simulink model "HorizontalClosedLoop"  (R2026b)
settings: Solver=FixedStepDiscrete  StopTime=25  FixedStep=.0025
undefined symbols (not defined in the file): Official
libraries: slpidlib x7
(part 1 of 3)
settings Model: Creator=tyasukaw  LastModifiedBy=tyasukaw

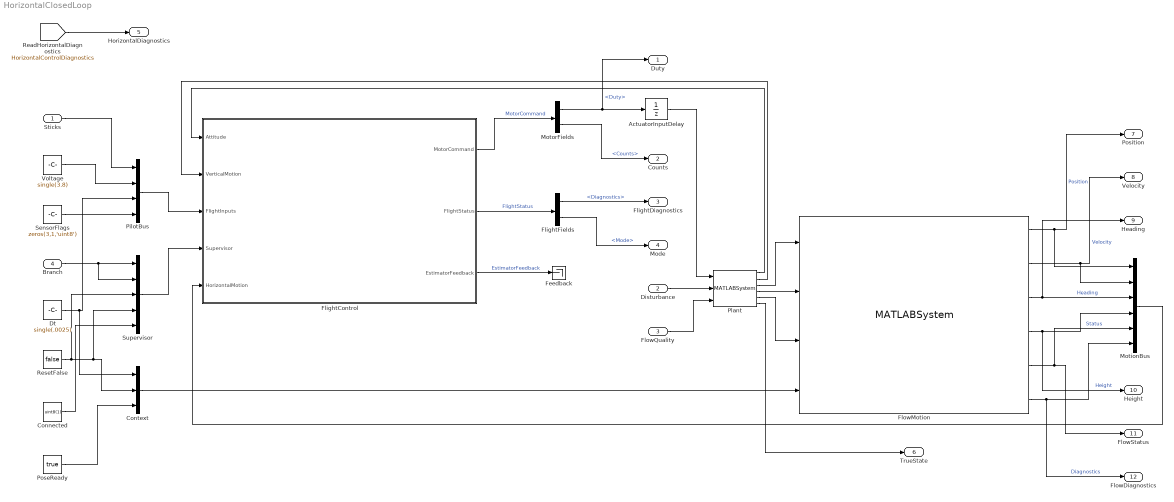
== system HorizontalClosedLoop ==
  Sticks : Inport  OutDataTypeStr=single  PortDimensions=6  SampleTime=.0025
  Disturbance : Inport  Port=2  OutDataTypeStr=single  PortDimensions=2  SampleTime=.0025
  FlowQuality : Inport  Port=3  OutDataTypeStr=uint16  SampleTime=.0025
  Branch : Inport  Port=4  OutDataTypeStr=uint8  SampleTime=.0025
  ActuatorInputDelay : UnitDelay  InitialCondition=zeros(4,1,'single')  SampleTime=.0025
  Connected : Constant  Value=uint8(1)
  Context : BusCreator  Inputs=3  OutDataTypeStr=Bus: HorizontalContextBus  NonVirtualBus=on
      settings: InheritFromInputs=off
  Dt : Constant  Value=single(.0025)
  Feedback : Terminator
  FlightControl : Subsystem  Description=最上位 Stateflow の指令と姿勢・高度を受け、離着陸、7 個の PID、モーター配分を計算します。出力は Duty・PWM Counts、飛行状態、次周期の推定器コンテキストです。状態ログもこの階層に含みます。
      mask help: 最上位 Stateflow の指令と姿勢・高度を受け、離着陸、7 個の PID、モーター配分を計算します。出力は Duty・PWM Counts、飛行状態、次周期の推定器コンテキストです。状態ログもこの階層に含みます。
      mask Display: disp('FlightControl');port_label('input',1,'Attitude');port_label('input',2,'VerticalMotion');port_label('input',3,'FlightInputs');port_label('input',4,'Supervisor');port_label('input',5,'HorizontalMotion');port_label('output',1,'MotorCommand');port_label('output',2,'FlightStatus');port_label('output',3,'EstimatorFeedback');
  FlightFields : BusSelector  OutputSignals=Diagnostics,Mode
  FlowMotion : MATLABSystem  Description=|  System=horizontal.FlowMotion  SampleTime=.0025  WindowSamples=8  XCountsPerRad=385  YCountsPerRad=385  MinQuality=25  MinHeightM=.12  MaxHeightM=1.0  MaxRangeAgeS=.15  MaxFlowAgeS=.025  MaxSampleGapS=.01  MaxGyroAgeS=.0075  MaxSpeedMps=1.5  MaxVerticalSpeedMps=2.0  MaxTiltDeg=25  VelocityTimeConstantS=.05  SimulateUsing=Code generation
      | %FLOWMOTION 概要：400 Hzの光学フロー・角速度を同一区間で集計し、
      |     % 50 Hzで水平速度と相対位置を推定します。局所Xは基準機首、Yは右。
      |     % 不良区間を速度ゼロに置き換えず、Statusで使用可否を公開します。
      mask Type: horizontal.FlowMotion
  MotionBus : BusCreator  Inputs=6  OutDataTypeStr=Bus: HorizontalMotionBus  NonVirtualBus=on
      settings: InheritFromInputs=off
  MotorFields : BusSelector  OutputSignals=Duty,Counts
  PilotBus : BusCreator  Inputs=4  OutDataTypeStr=Bus: HorizontalTestPilotBus  NonVirtualBus=on
      settings: InheritFromInputs=off
  Plant : MATLABSystem  System=horizontaltest.Plant  SampleTime=.0025  HoverDuty=.659  MotorLagS=.04  LinearDampingPerS=.5  TorqueAccelPerCount=.15  AngularDampingPerS=4  RangeDelayS=.035  FlowScale=1  GyroDelayS=0  HeadingDriftDegps=0  SimulateUsing=Code generation
      mask Type: horizontaltest.Plant
  PoseReady : Constant  Value=true
  ResetFalse : Constant  Value=false
  SensorFlags : Constant  Value=zeros(3,1,'uint8')
  Supervisor : BusCreator  Inputs=5  OutDataTypeStr=Bus: HorizontalTestSupervisorBus  NonVirtualBus=on
      settings: InheritFromInputs=off
  Voltage : Constant  Value=single(3.8)
  Duty : Outport
  Counts : Outport  Port=2
  FlightDiagnostics : Outport  Port=3
  Mode : Outport  Port=4
  HorizontalDiagnostics : Outport  Port=5
  TrueState : Outport  Port=6
  Position : Outport  Port=7
  Velocity : Outport  Port=8
  Heading : Outport  Port=9
  Height : Outport  Port=10
  FlowStatus : Outport  Port=11
  FlowDiagnostics : Outport  Port=12
  wires:
  Plant/6 -> TrueState/1
  [HorizontalControlDiagnostics] -> HorizontalDiagnostics/1
  FlightFields/2 -> Mode/1  "<Mode>"
  FlightFields/1 -> FlightDiagnostics/1  "<Diagnostics>"
  MotorFields/2 -> Counts/1  "<Counts>"
  FlowMotion/6 -> MotionBus/6, FlowDiagnostics/1  "Diagnostics"
  FlowMotion/5 -> MotionBus/5, FlowStatus/1  "Status"
  FlowMotion/4 -> MotionBus/4, Height/1  "Height"
  FlowMotion/3 -> MotionBus/3, Heading/1  "Heading"
  FlowMotion/2 -> MotionBus/2, Velocity/1  "Velocity"
  FlowMotion/1 -> MotionBus/1, Position/1  "Position"
  FlightControl/3(EstimatorFeedback) -> Feedback/1  "EstimatorFeedback"
  FlightControl/2(FlightStatus) -> FlightFields/1  "FlightStatus"
  PoseReady/1 -> Context/3
  Connected/1 -> Supervisor/5
  ResetFalse/1 -> Supervisor/4, Context/2, Supervisor/3
  Branch/1 -> Supervisor/1, Supervisor/2
  SensorFlags/1 -> PilotBus/4
  Dt/1 -> PilotBus/3, Context/1
  Voltage/1 -> PilotBus/2
  Sticks/1 -> PilotBus/1
  Context/1 -> FlowMotion/4
  Plant/5 -> FlowMotion/3
  Plant/4 -> FlowMotion/2
  Plant/3 -> FlowMotion/1
  FlowQuality/1 -> Plant/3
  Disturbance/1 -> Plant/2
  ActuatorInputDelay/1 -> Plant/1
  MotorFields/1 -> ActuatorInputDelay/1, Duty/1  "<Duty>"
  FlightControl/1(MotorCommand) -> MotorFields/1  "MotorCommand"
  MotionBus/1 -> FlightControl/5(HorizontalMotion)
  Supervisor/1 -> FlightControl/4(Supervisor)
  PilotBus/1 -> FlightControl/3(FlightInputs)
  Plant/2 -> FlightControl/2(VerticalMotion)
  Plant/1 -> FlightControl/1(Attitude)

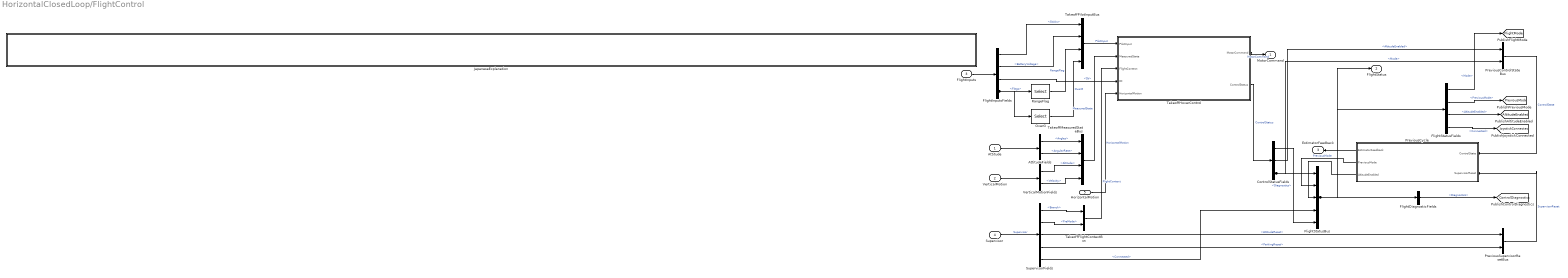
== system HorizontalClosedLoop/FlightControl ==
  Attitude : Inport
  VerticalMotion : Inport  Port=2
  FlightInputs : Inport  Port=3
  Supervisor : Inport  Port=4
  HorizontalMotion : Inport  Description=HorizontalMotion：水平推定・制御のデータと実行条件を選択・結合します。2軸の順序は局所X（基準機首）、Y（右）です。  Port=5  OutDataTypeStr=Bus: HorizontalMotionBus
  AttitudeFields : BusSelector  Description=AttitudeFields：バスから Angles,AngularRate を選びます。元のベクトルの成分順序は変更しません。  OutputSignals=Angles,AngularRate
  ControlStatusFields : BusSelector  Description=ControlStatusFields：バスから Diagnostics,AltitudeEnabled,Mode を選びます。元のベクトルの成分順序は変更しません。  OutputSignals=Diagnostics,AltitudeEnabled,Mode
  FlightDiagnosticFields : BusSelector  Description=FlightDiagnosticFields：バスから Diagnostics を選びます。元のベクトルの成分順序は変更しません。  OutputSignals=Diagnostics
  FlightInputsFields : BusSelector  Description=FlightInputsFields：バスから Sticks,BatteryVoltage,Dt,Flags を選びます。元のベクトルの成分順序は変更しません。  OutputSignals=Sticks,BatteryVoltage,Dt,Flags
  FlightStatusBus : BusCreator  Description=FlightStatusBus：異なる単位・型を持つ関連信号を名前付きバスにまとめます。入力線の信号名が項目名です。  Inputs=5
  FlightStatusFields : BusSelector  Description=FlightStatusFields：バスから Mode,PreviousMode,AltitudeEnabled,Connected を選びます。元のベクトルの成分順序は変更しません。  OutputSignals=Mode,PreviousMode,AltitudeEnabled,Connected
  JapaneseExplanation : Subsystem  Description=最上位 Stateflow の指令と姿勢・高度を受け、離着陸、7 個の PID、モーター配分を計算します。出力は Duty・PWM Counts、飛行状態、次周期の推定器コンテキストです。状態ログもこの階層に含みます。
      mask help: 最上位 Stateflow の指令と姿勢・高度を受け、離着陸、7 個の PID、モーター配分を計算します。出力は Duty・PWM Counts、飛行状態、次周期の推定器コンテキストです。状態ログもこの階層に含みます。
      mask Display: disp(sprintf('最上位 Stateflow の指令と姿勢・高度を受け、離着陸、7 個の PID、モーター配分を計算します。\n出力は Duty・PWM Counts、飛行状態、次周期の推定器コンテキストです。\n状態ログもこの階層に含みます。'));
  OverG : Selector  Description=OverG：必要なベクトル成分を選びます。選択位置は設定画面の Indices で確認します。  InputPortWidth=3  IndexOptions=Index vector (dialog)  Indices=1  OutputSizes=1
  PreviousControlStateBus : BusCreator  Description=PreviousControlStateBus：異なる単位・型を持つ関連信号を名前付きバスにまとめます。入力線の信号名が項目名です。  Inputs=2
  PreviousCycle : Subsystem  Description=前周期の推力・指令・モードなどを保持し、制御と次周期フィードバックへ渡します。Unit Delay は既存の更新順序を保つために必要です。
      mask help: 前周期の推力・指令・モードなどを保持し、制御と次周期フィードバックへ渡します。Unit Delay は既存の更新順序を保つために必要です。
      mask Display: disp('PreviousCycle');port_label('input',1,'ControlState');port_label('input',2,'SupervisorReset');port_label('output',1,'EstimatorFeedback');port_label('output',2,'PreviousMode');port_label('output',3,'AltitudeEnabled');
  PreviousSupervisorResetBus : BusCreator  Description=PreviousSupervisorResetBus：異なる単位・型を持つ関連信号を名前付きバスにまとめます。入力線の信号名が項目名です。  Inputs=2
  RangeFlag : Selector  Description=RangeFlag：必要なベクトル成分を選びます。選択位置は設定画面の Indices で確認します。  InputPortWidth=3  IndexOptions=Index vector (dialog)  Indices=2  OutputSizes=1
  SupervisorFields : BusSelector  Description=SupervisorFields：バスから Branch,PreMode,AttitudeReset,ParkingReset,Connected を選びます。元のベクトルの成分順序は変更しません。  OutputSignals=Branch,PreMode,AttitudeReset,ParkingReset,Connected
  TakeoffFlightContextBus : BusCreator  Description=TakeoffFlightContextBus：異なる単位・型を持つ関連信号を名前付きバスにまとめます。入力線の信号名が項目名です。  Inputs=2
  TakeoffHoverControl : Subsystem  Description=離着陸・高度制御・姿勢制御・角速度制御・モーター配分を機能別にまとめます。高度→速度、角度→角速度の二重ループを読みます。
      mask help: 離着陸・高度制御・姿勢制御・角速度制御・モーター配分を機能別にまとめます。高度→速度、角度→角速度の二重ループを読みます。
      mask Display: disp('TakeoffHoverControl');port_label('input',1,'PilotInput');port_label('input',2,'MeasuredState');port_label('input',3,'FlightContext');port_label('input',4,'Dt');port_label('input',5,'HorizontalMotion');port_label('output',1,'MotorCommand');port_label('output',2,'ControlStatus');
  TakeoffMeasuredStateBus : BusCreator  Description=TakeoffMeasuredStateBus：異なる単位・型を持つ関連信号を名前付きバスにまとめます。入力線の信号名が項目名です。  Inputs=4
  TakeoffPilotInputBus : BusCreator  Description=TakeoffPilotInputBus：異なる単位・型を持つ関連信号を名前付きバスにまとめます。入力線の信号名が項目名です。  Inputs=4
  VerticalMotionFields : BusSelector  Description=VerticalMotionFields：バスから Altitude,Velocity を選びます。元のベクトルの成分順序は変更しません。  OutputSignals=Altitude,Velocity
  MotorCommand : Outport
  FlightStatus : Outport  Port=2
  EstimatorFeedback : Outport  Port=3
  tag scope: AltitudeEnabled=global, ControlDiagnostics=global, FlightMode=global, JoystickConnected=global, PreviousMode=global
  wires:
  PreviousControlStateBus/1 -> PreviousCycle/1(ControlState)  "ControlState"
  FlightStatusFields/3 -> [AltitudeEnabled]  "<AltitudeEnabled>"
  PreviousCycle/1(EstimatorFeedback) -> EstimatorFeedback/1
  PreviousCycle/2(PreviousMode) -> FlightStatusBus/2  "PreviousMode"
  FlightStatusFields/1 -> [FlightMode]  "<Mode>"
  PreviousCycle/3(AltitudeEnabled) -> FlightStatusBus/3
  FlightStatusFields/2 -> [PreviousMode]  "<PreviousMode>"
  FlightStatusBus/1 -> FlightStatusFields/1, FlightDiagnosticFields/1, FlightStatus/1
  ControlStatusFields/3 -> FlightStatusBus/1, PreviousControlStateBus/2  "<Mode>"
  ControlStatusFields/1 -> FlightStatusBus/5  "<Diagnostics>"
  TakeoffHoverControl/1(MotorCommand) -> MotorCommand/1  "MotorCommand"
  HorizontalMotion/1 -> TakeoffHoverControl/5(HorizontalMotion)  "HorizontalMotion"
  TakeoffMeasuredStateBus/1 -> TakeoffHoverControl/2(MeasuredState)  "MeasuredState"
  TakeoffFlightContextBus/1 -> TakeoffHoverControl/3(FlightContext)  "FlightContext"
  TakeoffPilotInputBus/1 -> TakeoffHoverControl/1(PilotInput)  "PilotInput"
  SupervisorFields/5 -> FlightStatusBus/4  "<Connected>"
  SupervisorFields/4 -> PreviousSupervisorResetBus/2  "<ParkingReset>"
  SupervisorFields/3 -> PreviousSupervisorResetBus/1  "<AttitudeReset>"
  PreviousSupervisorResetBus/1 -> PreviousCycle/2(SupervisorReset)  "SupervisorReset"
  SupervisorFields/2 -> TakeoffFlightContextBus/2  "<PreMode>"
  SupervisorFields/1 -> TakeoffFlightContextBus/1  "<Branch>"
  TakeoffHoverControl/2(ControlStatus) -> ControlStatusFields/1  "ControlStatus"
  AttitudeFields/2 -> TakeoffMeasuredStateBus/2  "<AngularRate>"
  AttitudeFields/1 -> TakeoffMeasuredStateBus/1  "<Angles>"
  VerticalMotionFields/1 -> TakeoffMeasuredStateBus/3  "<Altitude>"
  OverG/1 -> TakeoffPilotInputBus/4  "OverG"
  RangeFlag/1 -> TakeoffPilotInputBus/3  "RangeFlag"
  VerticalMotionFields/2 -> TakeoffMeasuredStateBus/4  "<Velocity>"
  FlightInputsFields/2 -> TakeoffPilotInputBus/2  "<BatteryVoltage>"
  FlightInputsFields/4 -> OverG/1, RangeFlag/1  "<Flags>"
  FlightInputsFields/1 -> TakeoffPilotInputBus/1  "<Sticks>"
  FlightStatusFields/4 -> [JoystickConnected]  "<Connected>"
  FlightInputsFields/3 -> TakeoffHoverControl/4(Dt)  "<Dt>"
  FlightInputs/1 -> FlightInputsFields/1
  FlightDiagnosticFields/1 -> [ControlDiagnostics]  "<Diagnostics>"
  Attitude/1 -> AttitudeFields/1
  ControlStatusFields/2 -> PreviousControlStateBus/1  "<AltitudeEnabled>"
  VerticalMotion/1 -> VerticalMotionFields/1
  Supervisor/1 -> SupervisorFields/1  "Supervisor"

== system HorizontalClosedLoop/FlightControl/JapaneseExplanation ==

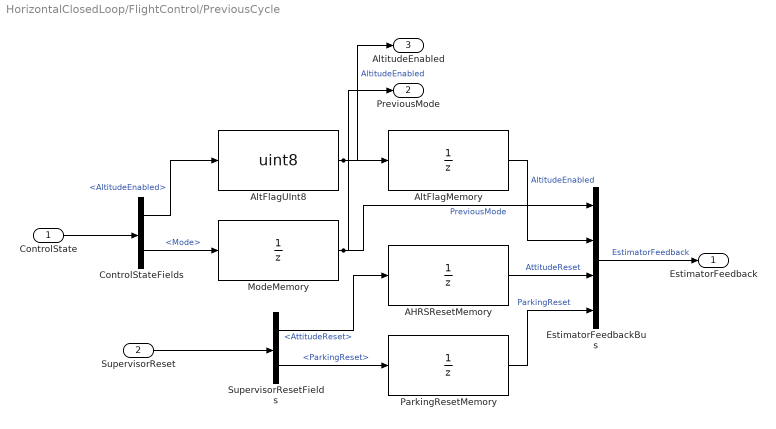
== system HorizontalClosedLoop/FlightControl/PreviousCycle ==
  ControlState : Inport
  SupervisorReset : Inport  Port=2
  AHRSResetMemory : UnitDelay  Description=AHRSResetMemory：前周期の値を保持して出力します。更新順序と状態保持に必要な 1 周期遅延です。初期値 false、周期 Official.Step 秒。  InitialCondition=false  SampleTime=Official.Step
  AltFlagMemory : UnitDelay  Description=AltFlagMemory：前周期の値を保持して出力します。更新順序と状態保持に必要な 1 周期遅延です。初期値 uint8(0)、周期 Official.Step 秒。  InitialCondition=uint8(0)  SampleTime=Official.Step
  AltFlagUInt8 : DataTypeConversion  Description=AltFlagUInt8：後段のバス・演算に合わせて uint8 型へ変換します。  OutDataTypeStr=uint8  SaturateOnIntegerOverflow=off  RndMeth=Floor
  ControlStateFields : BusSelector  Description=ControlStateFields：バスから AltitudeEnabled,Mode を選びます。元のベクトルの成分順序は変更しません。  OutputSignals=AltitudeEnabled,Mode
  EstimatorFeedbackBus : BusCreator  Description=EstimatorFeedbackBus：異なる単位・型を持つ関連信号を名前付きバスにまとめます。入力線の信号名が項目名です。  Inputs=4
  ModeMemory : UnitDelay  Description=ModeMemory：前周期の値を保持して出力します。更新順序と状態保持に必要な 1 周期遅延です。初期値 uint8(0)、周期 Official.Step 秒。  InitialCondition=uint8(0)  SampleTime=Official.Step
  ParkingResetMemory : UnitDelay  Description=ParkingResetMemory：前周期の値を保持して出力します。更新順序と状態保持に必要な 1 周期遅延です。初期値 false、周期 Official.Step 秒。  InitialCondition=false  SampleTime=Official.Step
  SupervisorResetFields : BusSelector  Description=SupervisorResetFields：バスから AttitudeReset,ParkingReset を選びます。元のベクトルの成分順序は変更しません。  OutputSignals=AttitudeReset,ParkingReset
  EstimatorFeedback : Outport
  PreviousMode : Outport  Port=2
  AltitudeEnabled : Outport  Port=3
  wires:
  AHRSResetMemory/1 -> EstimatorFeedbackBus/3  "AttitudeReset"
  EstimatorFeedbackBus/1 -> EstimatorFeedback/1  "EstimatorFeedback"
  AltFlagUInt8/1 -> AltitudeEnabled/1, AltFlagMemory/1  "AltitudeEnabled"
  ParkingResetMemory/1 -> EstimatorFeedbackBus/4  "ParkingReset"
  SupervisorResetFields/2 -> ParkingResetMemory/1  "<ParkingReset>"
  ControlStateFields/2 -> ModeMemory/1  "<Mode>"
  ControlState/1 -> ControlStateFields/1
  SupervisorReset/1 -> SupervisorResetFields/1
  ModeMemory/1 -> PreviousMode/1, EstimatorFeedbackBus/1  "PreviousMode"
  AltFlagMemory/1 -> EstimatorFeedbackBus/2  "AltitudeEnabled"
  SupervisorResetFields/1 -> AHRSResetMemory/1  "<AttitudeReset>"
  ControlStateFields/1 -> AltFlagUInt8/1  "<AltitudeEnabled>"

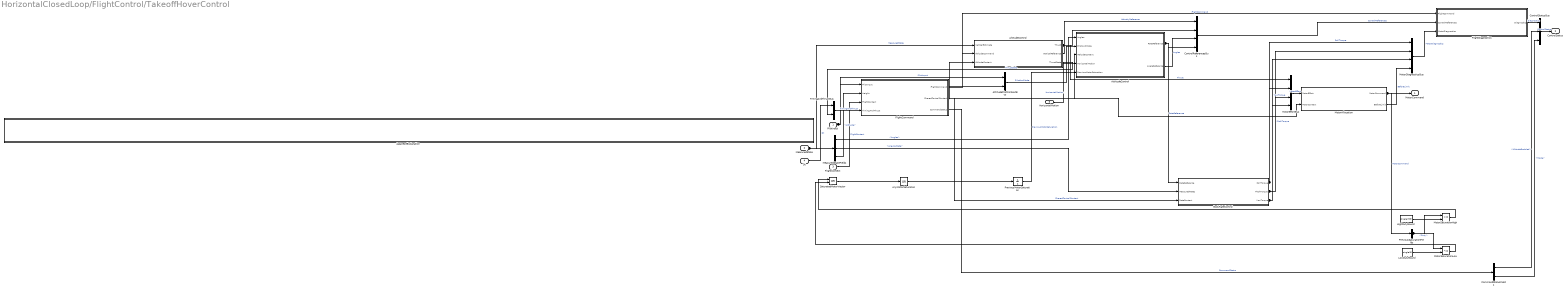
== system HorizontalClosedLoop/FlightControl/TakeoffHoverControl ==
  PilotInput : Inport
  MeasuredState : Inport  Port=2
  FlightContext : Inport  Port=3
  Dt : Inport  Port=4
  HorizontalMotion : Inport  Description=HorizontalMotion：水平推定・制御のデータと実行条件を選択・結合します。2軸の順序は局所X（基準機首）、Y（右）です。  Port=5  OutDataTypeStr=Bus: HorizontalMotionBus
  AltitudeControl : Subsystem  Description=高度誤差を高度 PID で目標鉛直速度へ変換し、鉛直速度 PID で共通推力を補正します。自動高度と着陸降下を選び、平滑化と推力制限を行います。
      mask help: 高度誤差を高度 PID で目標鉛直速度へ変換し、鉛直速度 PID で共通推力を補正します。自動高度と着陸降下を選び、平滑化と推力制限を行います。
      mask Display: disp('AltitudeControl');port_label('input',1,'VerticalEstimate');port_label('input',2,'AltitudeCommand');port_label('input',3,'AltitudeContext');port_label('output',1,'Thrust');port_label('output',2,'VerticalReference');port_label('output',3,'ThrustState');
  AnyMotorSaturation : Logic  Description=AnyMotorSaturation：水平推定・制御のデータと実行条件を選択・結合します。2軸の順序は局所X（基準機首）、Y（右）です。  Operator=OR  Inputs=1  IconShape=distinctive  AllPortsSameDT=off  OutDataTypeStr=boolean
  AttitudeControl : Subsystem  Description=Stabilize の Roll/Pitch 角度誤差を角度 PID へ渡して角速度目標を作ります。Sport は直接角速度目標を使い、Yaw の指令は角度ループを通しません。
      mask help: Stabilize の Roll/Pitch 角度誤差を角度 PID へ渡して角速度目標を作ります。Sport は直接角速度目標を使い、Yaw の指令は角度ループを通しません。
      mask Display: disp('AttitudeControl');port_label('input',1,'Angles');port_label('input',2,'PilotAndMode');port_label('input',3,'AttitudeContext');port_label('input',4,'HorizontalMotion');port_label('input',5,'PreviousMotorSaturation');port_label('output',1,'RateReference');port_label('output',2,'AngleReference');
  AttitudePilotContextBus : BusCreator  Description=AttitudePilotContextBus：異なる単位・型を持つ関連信号を名前付きバスにまとめます。入力線の信号名が項目名です。  Inputs=2
  BodyRateControl : Subsystem  Description=Roll/Pitch/Yaw の目標と推定角速度との差を各 PID で処理し、モーターに加える 3 軸の補正を作ります。角速度は機体 XYZ、rad/s です。
      mask help: Roll/Pitch/Yaw の目標と推定角速度との差を各 PID で処理し、モーターに加える 3 軸の補正を作ります。角速度は機体 XYZ、rad/s です。
      mask Display: disp('BodyRateControl');port_label('input',1,'RateReference');port_label('input',2,'MeasuredRates');port_label('input',3,'RateContext');port_label('output',1,'RollTorque');port_label('output',2,'PitchTorque');port_label('output',3,'YawTorque');
  CommandStatusFields : BusSelector  Description=CommandStatusFields：バスから AltitudeEnabled,Mode を選びます。元のベクトルの成分順序は変更しません。  OutputSignals=AltitudeEnabled,Mode
  ControlReferencesBus : BusCreator  Description=ControlReferencesBus：異なる単位・型を持つ関連信号を名前付きバスにまとめます。入力線の信号名が項目名です。  Inputs=4
  ControlStatusBus : BusCreator  Description=ControlStatusBus：異なる単位・型を持つ関連信号を名前付きバスにまとめます。入力線の信号名が項目名です。  Inputs=3
  FlightCommand : Subsystem  Description=スティック、高度目標、離着陸カウンター、共通推力とモードを決めます。低推力条件に応じた制御ループの許可・リセットも生成します。
      mask help: スティック、高度目標、離着陸カウンター、共通推力とモードを決めます。低推力条件に応じた制御ループの許可・リセットも生成します。
      mask Display: disp('FlightCommand');port_label('input',1,'PilotInput');port_label('input',2,'Height');port_label('input',3,'FlightContext');port_label('input',4,'TimingAndThrust');port_label('output',1,'FlightCommand');port_label('output',2,'SharedControlContext');port_label('output',3,'CommandStatus');
  FlightDiagnostics : Subsystem  Description=高度目標、推力、角度・角速度目標、3 軸補正、配分前値をログの既存 17 要素順序へまとめます。制御の判断は行いません。
      mask help: 高度目標、推力、角度・角速度目標、3 軸補正、配分前値をログの既存 17 要素順序へまとめます。制御の判断は行いません。
      mask Display: disp('FlightDiagnostics');port_label('input',1,'FlightCommand');port_label('input',2,'ControlReferences');port_label('input',3,'MotorDiagnostics');port_label('output',1,'Diagnostics');
  HighDutyBound : Constant  Description=HighDutyBound：水平推定・制御のデータと実行条件を選択・結合します。2軸の順序は局所X（基準機首）、Y（右）です。  Value=single(.95)
  JapaneseExplanation : Subsystem  Description=離着陸・高度制御・姿勢制御・角速度制御・モーター配分を機能別にまとめます。高度→速度、角度→角速度の二重ループを読みます。
      mask help: 離着陸・高度制御・姿勢制御・角速度制御・モーター配分を機能別にまとめます。高度→速度、角度→角速度の二重ループを読みます。
      mask Display: disp(sprintf('離着陸・高度制御・姿勢制御・角速度制御・モーター配分を機能別にまとめます。\n高度→速度、角度→角速度の二重ループを読みます。'));
  LowDutyBound : Constant  Description=LowDutyBound：水平推定・制御のデータと実行条件を選択・結合します。2軸の順序は局所X（基準機首）、Y（右）です。  Value=single(0)
  MeasuredStateFields : BusSelector  Description=MeasuredStateFields：バスから Angles,AngularRate,Altitude を選びます。元のベクトルの成分順序は変更しません。  OutputSignals=Angles,AngularRate,Altitude
  MotorAllocation : Subsystem  Description=共通推力と 3 軸の補正を [FR, FL, RR, RL] の 4 モーターへ配分します。3 ms 平滑化、Duty 0～0.95 の制限、floor(255*Duty) の量子化を行います。
      mask help: 共通推力と 3 軸の補正を [FR, FL, RR, RL] の 4 モーターへ配分します。3 ms 平滑化、Duty 0～0.95 の制限、floor(255*Duty) の量子化を行います。
      mask Display: disp('MotorAllocation');port_label('input',1,'MotorEffort');port_label('input',2,'MotorContext');port_label('output',1,'MotorCommand');port_label('output',2,'BeforeLimit');
  MotorDiagnosticsBus : BusCreator  Description=MotorDiagnosticsBus：異なる単位・型を持つ関連信号を名前付きバスにまとめます。入力線の信号名が項目名です。  Inputs=4
  MotorEffortBus : BusCreator  Description=MotorEffortBus：異なる単位・型を持つ関連信号を名前付きバスにまとめます。入力線の信号名が項目名です。  Inputs=4
  MotorSaturationHigh : RelationalOperator  Description=MotorSaturationHigh：水平推定・制御のデータと実行条件を選択・結合します。2軸の順序は局所X（基準機首）、Y（右）です。  OutDataTypeStr=boolean  RndMeth=Simplest  InputSameDT=off
  MotorSaturationLow : RelationalOperator  Description=MotorSaturationLow：水平推定・制御のデータと実行条件を選択・結合します。2軸の順序は局所X（基準機首）、Y（右）です。  Operator=<=  OutDataTypeStr=boolean  RndMeth=Simplest  InputSameDT=off
  PreviousMotorSaturation : UnitDelay  Description=PreviousMotorSaturation：水平推定・制御のデータと実行条件を選択・結合します。2軸の順序は局所X（基準機首）、Y（右）です。  InitialCondition=false  SampleTime=Official.Step
  PreviousSaturationFields : BusSelector  Description=PreviousSaturationFields：水平推定・制御のデータと実行条件を選択・結合します。2軸の順序は局所X（基準機首）、Y（右）です。  OutputSignals=Duty
  SaturatedMotorVector : Logic  Description=SaturatedMotorVector：水平推定・制御のデータと実行条件を選択・結合します。2軸の順序は局所X（基準機首）、Y（右）です。  Operator=OR  IconShape=distinctive  AllPortsSameDT=off  OutDataTypeStr=boolean
  TimingAndThrustBus : BusCreator  Description=TimingAndThrustBus：異なる単位・型を持つ関連信号を名前付きバスにまとめます。入力線の信号名が項目名です。  Inputs=2
  MotorCommand : Outport
  ControlStatus : Outport  Port=2
  wires:
  ControlStatusBus/1 -> ControlStatus/1  "ControlStatus"
  CommandStatusFields/2 -> ControlStatusBus/3  "<Mode>"
  FlightDiagnostics/1(Diagnostics) -> ControlStatusBus/1  "Diagnostics"
  PreviousSaturationFields/1 -> MotorSaturationLow/1, MotorSaturationHigh/1  "<Duty>"
  MotorAllocation/2(BeforeLimit) -> MotorDiagnosticsBus/4  "BeforeLimit"
  MotorAllocation/1(MotorCommand) -> MotorCommand/1, PreviousSaturationFields/1  "MotorCommand"
  MotorEffortBus/1 -> MotorAllocation/1(MotorEffort)  "MotorEffort"
  BodyRateControl/2(PitchTorque) -> MotorEffortBus/3, MotorDiagnosticsBus/2  "PitchTorque"
  BodyRateControl/1(RollTorque) -> MotorEffortBus/2, MotorDiagnosticsBus/1  "RollTorque"
  ControlReferencesBus/1 -> FlightDiagnostics/2(ControlReferences)  "ControlReferences"
  PreviousMotorSaturation/1 -> AttitudeControl/5(PreviousMotorSaturation)  "PreviousMotorSaturation"
  BodyRateControl/3(YawTorque) -> MotorEffortBus/4, MotorDiagnosticsBus/3  "YawTorque"
  LowDutyBound/1 -> MotorSaturationLow/2
  AttitudePilotContextBus/1 -> AttitudeControl/2(PilotAndMode)  "PilotAndMode"
  CommandStatusFields/1 -> ControlStatusBus/2  "<AltitudeEnabled>"
  AltitudeControl/3(ThrustState) -> TimingAndThrustBus/2  "ThrustState"
  MotorSaturationLow/1 -> SaturatedMotorVector/2
  AltitudeControl/1(Thrust) -> ControlReferencesBus/2, MotorEffortBus/1  "Thrust"
  AttitudeControl/2(AngleReference) -> ControlReferencesBus/3  "Angles"
  MotorSaturationHigh/1 -> SaturatedMotorVector/1
  FlightCommand/3(CommandStatus) -> CommandStatusFields/1  "CommandStatus"
  FlightCommand/2(SharedControlContext) -> AltitudeControl/3(AltitudeContext), AttitudePilotContextBus/2, AttitudeControl/3(AttitudeContext), MotorAllocation/2(MotorContext), BodyRateControl/3(RateContext)  "SharedControlContext"
  AltitudeControl/2(VerticalReference) -> ControlReferencesBus/1  "VelocityReference"
  AttitudeControl/1(RateReference) -> ControlReferencesBus/4, BodyRateControl/1(RateReference)  "RateReference"
  FlightCommand/1(FlightCommand) -> AltitudeControl/2(AltitudeCommand), FlightDiagnostics/1(FlightCommand)  "FlightCommand"
  MeasuredStateFields/2 -> BodyRateControl/2(MeasuredRates)  "<AngularRate>"
  MeasuredStateFields/1 -> AttitudeControl/1(Angles)  "<Angles>"
  TimingAndThrustBus/1 -> FlightCommand/4(TimingAndThrust)  "TimingAndThrust"
  Dt/1 -> TimingAndThrustBus/1  "Dt"
  MeasuredStateFields/3 -> FlightCommand/2(Height)  "<Altitude>"
  HorizontalMotion/1 -> AttitudeControl/4(HorizontalMotion)  "HorizontalMotion"
  MotorDiagnosticsBus/1 -> FlightDiagnostics/3(MotorDiagnostics)  "MotorDiagnostics"
  HighDutyBound/1 -> MotorSaturationHigh/2
  FlightContext/1 -> FlightCommand/3(FlightContext)  "FlightContext"
  SaturatedMotorVector/1 -> AnyMotorSaturation/1
  AnyMotorSaturation/1 -> PreviousMotorSaturation/1
  MeasuredState/1 -> MeasuredStateFields/1, AltitudeControl/1(VerticalEstimate)  "MeasuredState"
  PilotInput/1 -> FlightCommand/1(PilotInput), AttitudePilotContextBus/1  "PilotInput"

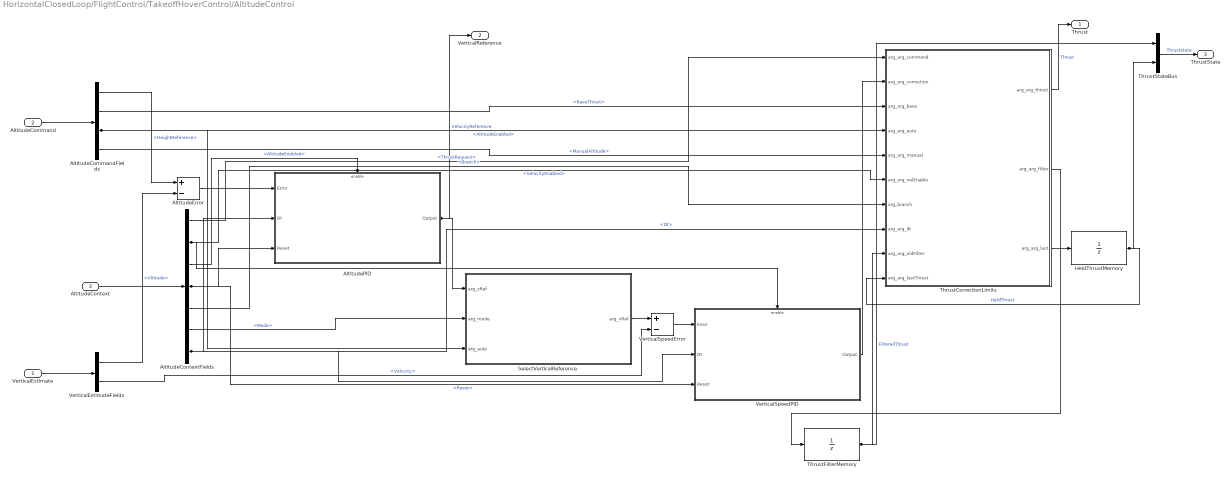
== system HorizontalClosedLoop/FlightControl/TakeoffHoverControl/AltitudeControl ==
  VerticalEstimate : Inport
  AltitudeCommand : Inport  Port=2
  AltitudeContext : Inport  Port=3
  AltitudeCommandFields : BusSelector  Description=AltitudeCommandFields：バスから HeightReference,BaseThrust,AltitudeEnabled,ManualAltitude を選びます。元のベクトルの成分順序は変更しません。  OutputSignals=HeightReference,BaseThrust,AltitudeEnabled,ManualAltitude
  AltitudeContextFields : BusSelector  Description=制御の実行・リセット条件と実測 dt を選びます。DedicatedPID 内部で前回誤差を保持するため、未使用の PreviousError は取り出しません。  OutputSignals=ThrustRequest,ControlContext.VelocityEnabled,ControlContext.AltitudeEnabled,ControlContext.Reset,FlightContext.Branch,Mode,Dt
  AltitudeError : Sum  Description=AltitudeError：入力を +- の符号で加減算します。ベクトルでは各成分に同じ演算を適用します。  Inputs=+-
  AltitudePID : Subsystem  Description=高度 PID：高度誤差→鉛直速度目標。Enabled subsystem が状態更新を許可し、低推力 Reset が積分・微分状態を初期化します。内部 DedicatedPID は Ideal・離散・台形積分/微分・外部 dt です。P=0.38、I=0.1、D=0.5、N=16。
      mask help: 高度 PID：高度誤差→鉛直速度目標。Enabled subsystem が状態更新を許可し、低推力 Reset が積分・微分状態を初期化します。内部 DedicatedPID は Ideal・離散・台形積分/微分・外部 dt です。P=0.38、I=0.1、D=0.5、N=16。
      mask Display: disp('AltitudePID');port_label('input',1,'Error');port_label('input',2,'Dt');port_label('input',3,'Reset');port_label('output',1,'Output');
  HeldThrustMemory : UnitDelay  Description=HeldThrustMemory：前周期の値を保持して出力します。更新順序と状態保持に必要な 1 周期遅延です。初期値 single(0)、周期 Official.Step 秒。  InitialCondition=single(0)  SampleTime=Official.Step
  SelectVerticalReference : MATLAB Function  Description=鉛直速度目標を選びます。Auto Altitude 時は高度 PID の目標を使い、手動高度で着陸中（Mode 5）のときだけ -0.15 の降下目標に切り替えます。  TreatAsAtomicUnit=on
  ThrustCorrectionLimits : MATLAB Function  Description=共通推力を決めます。鉛直速度 PID の補正を基準推力へ加え、10 ms で平滑化します。Auto Altitude 時は基準の 0.85～1.15 倍に制限し、指定された分岐では前回推力を保持します。  TreatAsAtomicUnit=on
  ThrustFilterMemory : UnitDelay  Description=ThrustFilterMemory：前周期の値を保持して出力します。更新順序と状態保持に必要な 1 周期遅延です。初期値 single(0)、周期 Official.Step 秒。  InitialCondition=single(0)  SampleTime=Official.Step
  ThrustStateBus : BusCreator  Description=ThrustStateBus：異なる単位・型を持つ関連信号を名前付きバスにまとめます。入力線の信号名が項目名です。  Inputs=2
  VerticalEstimateFields : BusSelector  Description=VerticalEstimateFields：バスから Altitude,Velocity を選びます。元のベクトルの成分順序は変更しません。  OutputSignals=Altitude,Velocity
  VerticalSpeedError : Sum  Description=VerticalSpeedError：入力を +- の符号で加減算します。ベクトルでは各成分に同じ演算を適用します。  Inputs=+-
  VerticalSpeedPID : Subsystem  Description=鉛直速度 PID：速度誤差→基準推力の補正。Enabled 境界・外部 Reset・実測 dt と既存係数を保持します。内部の DedicatedPID で係数を設定します。
      mask help: 鉛直速度 PID：速度誤差→基準推力の補正。Enabled 境界・外部 Reset・実測 dt と既存係数を保持します。内部の DedicatedPID で係数を設定します。
      mask Display: disp('VerticalSpeedPID');port_label('input',1,'Error');port_label('input',2,'Dt');port_label('input',3,'Reset');port_label('output',1,'Output');
  Thrust : Outport
  VerticalReference : Outport  Port=2
  ThrustState : Outport  Port=3
  wires:
  ThrustStateBus/1 -> ThrustState/1  "ThrustState"
  HeldThrustMemory/1 -> ThrustStateBus/2, ThrustCorrectionLimits/10(arg_arg_lastThrust)  "HeldThrust"
  ThrustCorrectionLimits/3(arg_arg_last) -> HeldThrustMemory/1
  ThrustCorrectionLimits/2(arg_arg_filter) -> ThrustFilterMemory/1
  ThrustCorrectionLimits/1(arg_arg_thrust) -> Thrust/1  "Thrust"
  ThrustFilterMemory/1 -> ThrustCorrectionLimits/9(arg_arg_oldFilter), ThrustStateBus/1  "FilteredThrust"
  VerticalSpeedPID/1(Output) -> ThrustCorrectionLimits/2(arg_arg_correction)
  VerticalSpeedError/1 -> VerticalSpeedPID/1(Error)
  AltitudeContextFields/7 -> AltitudePID/2(Dt), VerticalSpeedPID/2(Dt), ThrustCorrectionLimits/8(arg_arg_dt)  "<Dt>"
  AltitudeContextFields/6 -> SelectVerticalReference/2(arg_mode)  "<Mode>"
  AltitudeContextFields/5 -> ThrustCorrectionLimits/7(arg_branch)  "<Branch>"
  AltitudeContextFields/4 -> VerticalSpeedPID/3(Reset), AltitudePID/3(Reset)  "<Reset>"
  AltitudeContextFields/3 -> AltitudePID/Enable  "<AltitudeEnabled>"
  AltitudeContextFields/2 -> ThrustCorrectionLimits/6(arg_arg_velEnable), VerticalSpeedPID/Enable  "<VelocityEnabled>"
  SelectVerticalReference/1(arg_vRef) -> VerticalSpeedError/1
  AltitudeContextFields/1 -> ThrustCorrectionLimits/1(arg_arg_command)  "<ThrustRequest>"
  AltitudePID/1(Output) -> VerticalReference/1, SelectVerticalReference/1(arg_zRef)  "VelocityReference"
  AltitudeError/1 -> AltitudePID/1(Error)
  VerticalEstimateFields/2 -> VerticalSpeedError/2  "<Velocity>"
  VerticalEstimateFields/1 -> AltitudeError/2  "<Altitude>"
  AltitudeCommandFields/1 -> AltitudeError/1  "<HeightReference>"
  AltitudeCommandFields/3 -> ThrustCorrectionLimits/4(arg_arg_auto), SelectVerticalReference/3(arg_auto)  "<AltitudeEnabled>"
  AltitudeCommand/1 -> AltitudeCommandFields/1
  VerticalEstimate/1 -> VerticalEstimateFields/1
  AltitudeCommandFields/2 -> ThrustCorrectionLimits/3(arg_arg_base)  "<BaseThrust>"
  AltitudeCommandFields/4 -> ThrustCorrectionLimits/5(arg_arg_manual)  "<ManualAltitude>"
  AltitudeContext/1 -> AltitudeContextFields/1

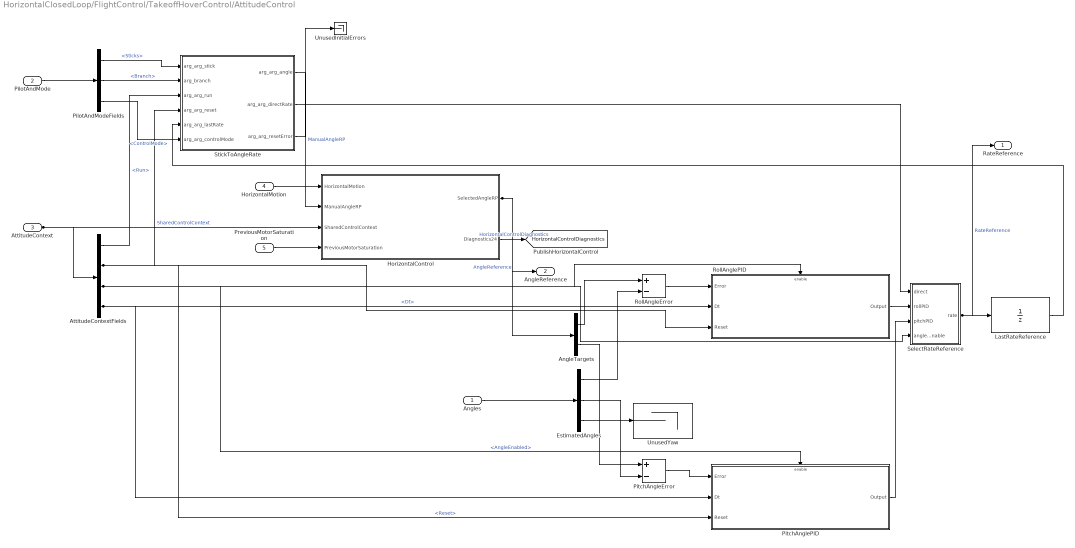
== system HorizontalClosedLoop/FlightControl/TakeoffHoverControl/AttitudeControl ==
  Angles : Inport
  PilotAndMode : Inport  Port=2
  AttitudeContext : Inport  Port=3
  HorizontalMotion : Inport  Description=HorizontalMotion：水平推定・制御のデータと実行条件を選択・結合します。2軸の順序は局所X（基準機首）、Y（右）です。  Port=4  OutDataTypeStr=Bus: HorizontalMotionBus
  PreviousMotorSaturation : Inport  Description=PreviousMotorSaturation：水平推定・制御のデータと実行条件を選択・結合します。2軸の順序は局所X（基準機首）、Y（右）です。  Port=5  OutDataTypeStr=boolean
  AngleTargets : Demux  Description=AngleTargets：ベクトルを元の成分順に分解します。個別の誤差や符号処理が必要な箇所で使います。  Outputs=2
  AttitudeContextFields : BusSelector  Description=AttitudeContextFields：バスから ControlContext.Run,ControlContext.Reset,ControlContext.AngleEnabled,Dt を選びます。元のベクトルの成分順序は変更しません。  OutputSignals=ControlContext.Run,ControlContext.Reset,ControlContext.AngleEnabled,Dt
  EstimatedAngles : Demux  Description=EstimatedAngles：ベクトルを元の成分順に分解します。個別の誤差や符号処理が必要な箇所で使います。  Outputs=3
  HorizontalControl : Subsystem  Description=HorizontalControl：水平推定・制御のデータと実行条件を選択・結合します。2軸の順序は局所X（基準機首）、Y（右）です。
      mask help: 水平制御：移動・減速・停止位置保持の速度目標、速度PI、姿勢目標への変換を行います。既存の姿勢・角速度PIDの前段です。
      mask Display: disp('HorizontalControl');port_label('input',1,'HorizontalMotion');port_label('input',2,'ManualAngleRP');port_label('input',3,'SharedControlContext');port_label('input',4,'PreviousMotorSaturation');port_label('output',1,'SelectedAngleRP');port_label('output',2,'Diagnostics24');
  LastRateReference : UnitDelay  Description=LastRateReference：前周期の値を保持して出力します。更新順序と状態保持に必要な 1 周期遅延です。初期値 zeros(3,1,'single')、周期 Official.Step 秒。  InitialCondition=zeros(3,1,'single')  SampleTime=Official.Step
  PilotAndModeFields : BusSelector  Description=PilotAndModeFields：バスから PilotInput.Sticks,SharedControlContext.FlightContext.Branch,SharedControlContext.ControlMode を選びます。元のベクトルの成分順序は変更しません。  OutputSignals=PilotInput.Sticks,SharedControlContext.FlightContext.Branch,SharedControlContext.ControlMode
  PitchAngleError : Sum  Description=PitchAngleError：入力を +- の符号で加減算します。ベクトルでは各成分に同じ演算を適用します。  Inputs=+-
  PitchAnglePID : Subsystem  Description=Pitch 角度 PID：角度誤差 [rad]→Pitch 角速度目標 [rad/s]。Stabilize 時の Enabled 境界と低推力 Reset を保ちます。
      mask help: Pitch 角度 PID：角度誤差 [rad]→Pitch 角速度目標 [rad/s]。Stabilize 時の Enabled 境界と低推力 Reset を保ちます。
      mask Display: disp('PitchAnglePID');port_label('input',1,'Error');port_label('input',2,'Dt');port_label('input',3,'Reset');port_label('output',1,'Output');
  RollAngleError : Sum  Description=RollAngleError：入力を +- の符号で加減算します。ベクトルでは各成分に同じ演算を適用します。  Inputs=+-
  RollAnglePID : Subsystem  Description=Roll 角度 PID：角度誤差 [rad]→Roll 角速度目標 [rad/s]。Stabilize 時の Enabled 境界と低推力 Reset を保ちます。
      mask help: Roll 角度 PID：角度誤差 [rad]→Roll 角速度目標 [rad/s]。Stabilize 時の Enabled 境界と低推力 Reset を保ちます。
      mask Display: disp('RollAnglePID');port_label('input',1,'Error');port_label('input',2,'Dt');port_label('input',3,'Reset');port_label('output',1,'Output');
  SelectRateReference : MATLAB Function  Description=角速度 PID の目標 [Roll, Pitch, Yaw] を選びます。Stabilize で角度制御が有効なときだけ Roll/Pitch を角度 PID の出力へ置換し、Yaw と Sport の直接角速度目標はそのまま使います。  TreatAsAtomicUnit=on
  StickToAngleRate : MATLAB Function  Description=操縦スティックから角度・角速度目標を作ります。Stabilize は Roll/Pitch ±30°、Sport は非線形な角速度指令、Yaw は角速度指令です。低推力リセット時に中立値を記憶します。  TreatAsAtomicUnit=on
  UnusedInitialErrors : Terminator
      settings: Description=操縦指令の既存関数が返す初期誤差を終端します。DedicatedPID の Reset により内部誤差を管理します。
  UnusedYaw : Terminator
      settings: Description=UnusedYaw：使用しない観測出力をここで終端します。接続された制御信号を変更しません。
  RateReference : Outport
  AngleReference : Outport  Port=2
  tag scope: HorizontalControlDiagnostics=global
  wires:
  LastRateReference/1 -> StickToAngleRate/5(arg_arg_lastRate)
  PitchAnglePID/1(Output) -> SelectRateReference/3(pitchPID)
  PitchAngleError/1 -> PitchAnglePID/1(Error)
  RollAngleError/1 -> RollAnglePID/1(Error)
  EstimatedAngles/3 -> UnusedYaw/1
  EstimatedAngles/1 -> RollAngleError/2
  SelectRateReference/1(rate) -> RateReference/1, LastRateReference/1  "RateReference"
  AngleTargets/2 -> PitchAngleError/1
  AngleTargets/1 -> RollAngleError/1
  HorizontalControl/2(Diagnostics24) -> [HorizontalControlDiagnostics]  "HorizontalControlDiagnostics"
  HorizontalControl/1(SelectedAngleRP) -> AngleTargets/1, AngleReference/1  "AngleReference"
  PreviousMotorSaturation/1 -> HorizontalControl/4(PreviousMotorSaturation)
  RollAnglePID/1(Output) -> SelectRateReference/2(rollPID)
  HorizontalMotion/1 -> HorizontalControl/1(HorizontalMotion)
  EstimatedAngles/2 -> PitchAngleError/2
  StickToAngleRate/3(arg_arg_resetError) -> UnusedInitialErrors/1
  StickToAngleRate/2(arg_arg_directRate) -> SelectRateReference/1(direct)
  StickToAngleRate/1(arg_arg_angle) -> HorizontalControl/2(ManualAngleRP)  "ManualAngleRP"
  AttitudeContextFields/1 -> StickToAngleRate/3(arg_arg_run)  "<Run>"
  AttitudeContextFields/3 -> RollAnglePID/Enable, SelectRateReference/4(angleEnable), PitchAnglePID/Enable  "<AngleEnabled>"
  PilotAndModeFields/2 -> StickToAngleRate/2(arg_branch)  "<Branch>"
  PilotAndModeFields/1 -> StickToAngleRate/1(arg_arg_stick)  "<Sticks>"
  PilotAndModeFields/3 -> StickToAngleRate/6(arg_arg_controlMode)  "<ControlMode>"
  PilotAndMode/1 -> PilotAndModeFields/1
  AttitudeContextFields/4 -> RollAnglePID/2(Dt), PitchAnglePID/2(Dt)  "<Dt>"
  AttitudeContext/1 -> AttitudeContextFields/1, HorizontalControl/3(SharedControlContext)  "SharedControlContext"
  AttitudeContextFields/2 -> StickToAngleRate/4(arg_arg_reset), PitchAnglePID/3(Reset), RollAnglePID/3(Reset)  "<Reset>"
  Angles/1 -> EstimatedAngles/1

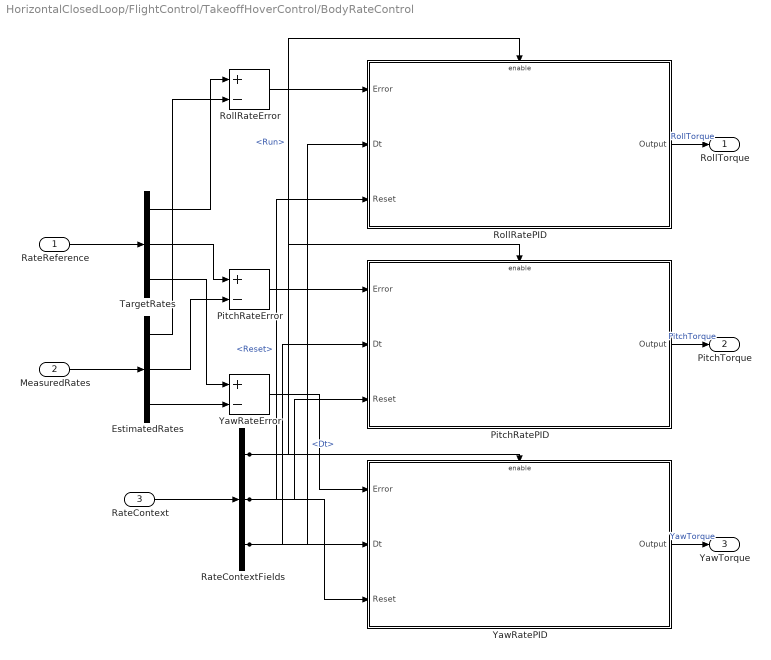
== system HorizontalClosedLoop/FlightControl/TakeoffHoverControl/BodyRateControl ==
  RateReference : Inport
  MeasuredRates : Inport  Port=2
  RateContext : Inport  Port=3
  EstimatedRates : Demux  Description=EstimatedRates：ベクトルを元の成分順に分解します。個別の誤差や符号処理が必要な箇所で使います。  Outputs=3
  PitchRateError : Sum  Description=PitchRateError：入力を +- の符号で加減算します。ベクトルでは各成分に同じ演算を適用します。  Inputs=+-
  PitchRatePID : Subsystem  Description=Pitch 角速度 PID：角速度誤差 [rad/s]→Pitch のモーター補正。積分状態は Enable と Reset で管理し、実測 dt を入力します。
      mask help: Pitch 角速度 PID：角速度誤差 [rad/s]→Pitch のモーター補正。積分状態は Enable と Reset で管理し、実測 dt を入力します。
      mask Display: disp('PitchRatePID');port_label('input',1,'Error');port_label('input',2,'Dt');port_label('input',3,'Reset');port_label('output',1,'Output');
  RateContextFields : BusSelector  Description=制御の実行・リセット条件と実測 dt を選びます。DedicatedPID 内部で前回誤差を保持するため、未使用の PreviousError は取り出しません。  OutputSignals=ControlContext.Run,ControlContext.Reset,Dt
  RollRateError : Sum  Description=RollRateError：入力を +- の符号で加減算します。ベクトルでは各成分に同じ演算を適用します。  Inputs=+-
  RollRatePID : Subsystem  Description=Roll 角速度 PID：角速度誤差 [rad/s]→Roll のモーター補正。積分状態は Enable と Reset で管理し、実測 dt を入力します。
      mask help: Roll 角速度 PID：角速度誤差 [rad/s]→Roll のモーター補正。積分状態は Enable と Reset で管理し、実測 dt を入力します。
      mask Display: disp('RollRatePID');port_label('input',1,'Error');port_label('input',2,'Dt');port_label('input',3,'Reset');port_label('output',1,'Output');
  TargetRates : Demux  Description=TargetRates：ベクトルを元の成分順に分解します。個別の誤差や符号処理が必要な箇所で使います。  Outputs=3
  YawRateError : Sum  Description=YawRateError：入力を +- の符号で加減算します。ベクトルでは各成分に同じ演算を適用します。  Inputs=+-
  YawRatePID : Subsystem  Description=Yaw 角速度 PID：角速度誤差 [rad/s]→Yaw のモーター補正。Yaw の絶対角度制御は行わず、スティックの角速度目標を使います。
      mask help: Yaw 角速度 PID：角速度誤差 [rad/s]→Yaw のモーター補正。Yaw の絶対角度制御は行わず、スティックの角速度目標を使います。
      mask Display: disp('YawRatePID');port_label('input',1,'Error');port_label('input',2,'Dt');port_label('input',3,'Reset');port_label('output',1,'Output');
  RollTorque : Outport
  PitchTorque : Outport  Port=2
  YawTorque : Outport  Port=3
  wires:
  YawRatePID/1(Output) -> YawTorque/1  "YawTorque"
  PitchRatePID/1(Output) -> PitchTorque/1  "PitchTorque"
  RollRatePID/1(Output) -> RollTorque/1  "RollTorque"
  RateContextFields/3 -> PitchRatePID/2(Dt), RollRatePID/2(Dt), YawRatePID/2(Dt)  "<Dt>"
  RateContextFields/2 -> YawRatePID/3(Reset), RollRatePID/3(Reset), PitchRatePID/3(Reset)  "<Reset>"
  RateContextFields/1 -> PitchRatePID/Enable, RollRatePID/Enable, YawRatePID/Enable  "<Run>"
  YawRateError/1 -> YawRatePID/1(Error)
  PitchRateError/1 -> PitchRatePID/1(Error)
  RollRateError/1 -> RollRatePID/1(Error)
  RateContext/1 -> RateContextFields/1
  EstimatedRates/1 -> RollRateError/2
  EstimatedRates/3 -> YawRateError/2
  TargetRates/2 -> PitchRateError/1
  TargetRates/1 -> RollRateError/1
  TargetRates/3 -> YawRateError/1
  RateReference/1 -> TargetRates/1
  MeasuredRates/1 -> EstimatedRates/1
  EstimatedRates/2 -> PitchRateError/2

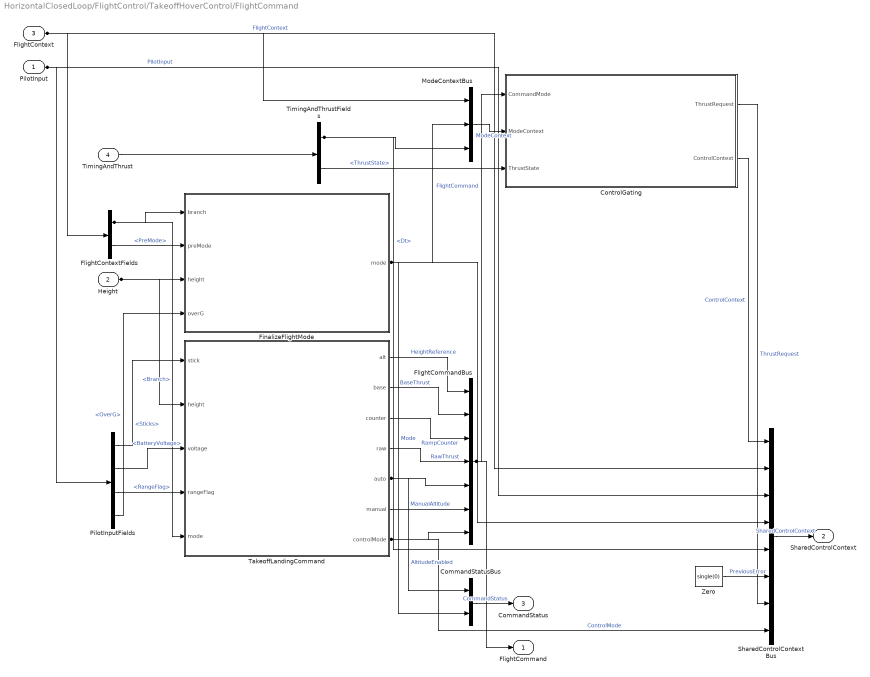
== system HorizontalClosedLoop/FlightControl/TakeoffHoverControl/FlightCommand ==
  PilotInput : Inport
  Height : Inport  Port=2
  FlightContext : Inport  Port=3
  TimingAndThrust : Inport  Port=4
  CommandStatusBus : BusCreator  Description=CommandStatusBus：異なる単位・型を持つ関連信号を名前付きバスにまとめます。入力線の信号名が項目名です。  Inputs=2
  ControlGating : Subsystem  Description=共通推力と飛行分岐から、全体・高度・角度・鉛直速度 PID の実行条件とリセットを決めます。制御の積分状態を校正・待機中に進めないための条件です。
      mask help: 共通推力と飛行分岐から、全体・高度・角度・鉛直速度 PID の実行条件とリセットを決めます。制御の積分状態を校正・待機中に進めないための条件です。
      mask Display: disp('ControlGating');port_label('input',1,'CommandMode');port_label('input',2,'ModeContext');port_label('input',3,'ThrustState');port_label('output',1,'ThrustRequest');port_label('output',2,'ControlContext');
  FinalizeFlightMode : Stateflow chart  Description=離着陸カウンターと制御状態から、周期末のモード・接続状態などを確定します。次周期に渡すモードと最上位の分岐を区別します。  TreatAsAtomicUnit=on
      mask help: 離着陸カウンターと制御状態から、周期末のモード・接続状態などを確定します。次周期に渡すモードと最上位の分岐を区別します。
  FlightCommandBus : BusCreator  Description=FlightCommandBus：異なる単位・型を持つ関連信号を名前付きバスにまとめます。入力線の信号名が項目名です。  Inputs=7
  FlightContextFields : BusSelector  Description=FlightContextFields：バスから Branch,PreMode を選びます。元のベクトルの成分順序は変更しません。  OutputSignals=Branch,PreMode
  ModeContextBus : BusCreator  Description=ModeContextBus：異なる単位・型を持つ関連信号を名前付きバスにまとめます。入力線の信号名が項目名です。  Inputs=3
  PilotInputFields : BusSelector  Description=PilotInputFields：バスから Sticks,BatteryVoltage,RangeFlag,OverG を選びます。元のベクトルの成分順序は変更しません。  OutputSignals=Sticks,BatteryVoltage,RangeFlag,OverG
  SharedControlContextBus : BusCreator  Description=SharedControlContextBus：異なる単位・型を持つ関連信号を名前付きバスにまとめます。入力線の信号名が項目名です。  Inputs=8
  TakeoffLandingCommand : Stateflow chart  Description=離陸・着陸、0.5 m の初期高度目標、0.05～1.8 m の高さ設定、基準推力と電圧トリムを状態として管理する Stateflow です。  TreatAsAtomicUnit=on
      mask help: 離陸・着陸、0.5 m の初期高度目標、0.05～1.8 m の高さ設定、基準推力と電圧トリムを状態として管理する Stateflow です。
  TimingAndThrustFields : BusSelector  Description=TimingAndThrustFields：バスから Dt,ThrustState を選びます。元のベクトルの成分順序は変更しません。  OutputSignals=Dt,ThrustState
  Zero : Constant  Description=Zero：固定値 single(0) を出力します。意味と単位は親の機能説明と信号名を参照します。  Value=single(0)
  FlightCommand : Outport
  SharedControlContext : Outport  Port=2
  CommandStatus : Outport  Port=3
  wires:
  SharedControlContextBus/1 -> SharedControlContext/1  "SharedControlContext"
  Zero/1 -> SharedControlContextBus/6  "PreviousError"
  CommandStatusBus/1 -> CommandStatus/1  "CommandStatus"
  FlightCommandBus/1 -> FlightCommand/1, ControlGating/1(CommandMode)  "FlightCommand"
  TakeoffLandingCommand/6(manual) -> FlightCommandBus/6  "ManualAltitude"
  TakeoffLandingCommand/3(counter) -> FlightCommandBus/3  "RampCounter"
  TakeoffLandingCommand/2(base) -> FlightCommandBus/2  "BaseThrust"
  TakeoffLandingCommand/1(alt) -> FlightCommandBus/1  "HeightReference"
  ControlGating/1(ThrustRequest) -> SharedControlContextBus/7  "ThrustRequest"
  FinalizeFlightMode/1(mode) -> ModeContextBus/2, CommandStatusBus/2, SharedControlContextBus/4  "Mode"
  TimingAndThrustFields/2 -> ControlGating/3(ThrustState)  "<ThrustState>"
  TimingAndThrustFields/1 -> ModeContextBus/3, SharedControlContextBus/5  "<Dt>"
  PilotInputFields/4 -> FinalizeFlightMode/4(overG)  "<OverG>"
  PilotInputFields/3 -> TakeoffLandingCommand/4(rangeFlag)  "<RangeFlag>"
  PilotInputFields/2 -> TakeoffLandingCommand/3(voltage)  "<BatteryVoltage>"
  FlightContextFields/2 -> FinalizeFlightMode/2(preMode)  "<PreMode>"
  TakeoffLandingCommand/5(auto) -> CommandStatusBus/1, FlightCommandBus/5  "AltitudeEnabled"
  PilotInputFields/1 -> TakeoffLandingCommand/1(stick)  "<Sticks>"
  FlightContextFields/1 -> FinalizeFlightMode/1(branch), TakeoffLandingCommand/5(mode)  "<Branch>"
  TakeoffLandingCommand/4(raw) -> FlightCommandBus/4  "RawThrust"
  FlightContext/1 -> FlightContextFields/1, SharedControlContextBus/2, ModeContextBus/1  "FlightContext"
  TakeoffLandingCommand/7(controlMode) -> FlightCommandBus/7, SharedControlContextBus/8  "ControlMode"
  PilotInput/1 -> PilotInputFields/1, SharedControlContextBus/3  "PilotInput"
  ControlGating/2(ControlContext) -> SharedControlContextBus/1  "ControlContext"
  TimingAndThrust/1 -> TimingAndThrustFields/1
  Height/1 -> TakeoffLandingCommand/2(height), FinalizeFlightMode/3(height)
  ModeContextBus/1 -> ControlGating/2(ModeContext)  "ModeContext"

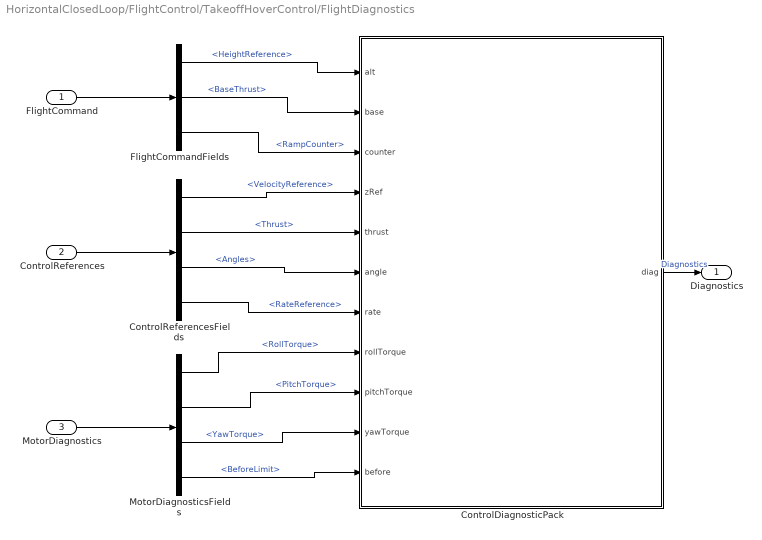
== system HorizontalClosedLoop/FlightControl/TakeoffHoverControl/FlightDiagnostics ==
  FlightCommand : Inport
  ControlReferences : Inport  Port=2
  MotorDiagnostics : Inport  Port=3
  ControlDiagnosticPack : MATLAB Function  Description=制御内部の観測値を 17 要素の single ベクトルにまとめます。ログの項目順は [高度制御状態; 基準推力; 離陸カウンター; 高度目標; 推力; 角度目標2; 角速度目標3; 軸補正3; 配分前モーター値4] です。制御判断は行いません。  TreatAsAtomicUnit=on
  ControlReferencesFields : BusSelector  Description=ControlReferencesFields：バスから VelocityReference,Thrust,Angles,RateReference を選びます。元のベクトルの成分順序は変更しません。  OutputSignals=VelocityReference,Thrust,Angles,RateReference
  FlightCommandFields : BusSelector  Description=FlightCommandFields：バスから HeightReference,BaseThrust,RampCounter を選びます。元のベクトルの成分順序は変更しません。  OutputSignals=HeightReference,BaseThrust,RampCounter
  MotorDiagnosticsFields : BusSelector  Description=MotorDiagnosticsFields：バスから RollTorque,PitchTorque,YawTorque,BeforeLimit を選びます。元のベクトルの成分順序は変更しません。  OutputSignals=RollTorque,PitchTorque,YawTorque,BeforeLimit
  Diagnostics : Outport
  wires:
  ControlDiagnosticPack/1(diag) -> Diagnostics/1  "Diagnostics"
  MotorDiagnosticsFields/4 -> ControlDiagnosticPack/11(before)  "<BeforeLimit>"
  MotorDiagnosticsFields/3 -> ControlDiagnosticPack/10(yawTorque)  "<YawTorque>"
  MotorDiagnosticsFields/2 -> ControlDiagnosticPack/9(pitchTorque)  "<PitchTorque>"
  MotorDiagnosticsFields/1 -> ControlDiagnosticPack/8(rollTorque)  "<RollTorque>"
  ControlReferencesFields/4 -> ControlDiagnosticPack/7(rate)  "<RateReference>"
  ControlReferencesFields/3 -> ControlDiagnosticPack/6(angle)  "<Angles>"
  ControlReferencesFields/2 -> ControlDiagnosticPack/5(thrust)  "<Thrust>"
  FlightCommandFields/3 -> ControlDiagnosticPack/3(counter)  "<RampCounter>"
  ControlReferencesFields/1 -> ControlDiagnosticPack/4(zRef)  "<VelocityReference>"
  FlightCommandFields/2 -> ControlDiagnosticPack/2(base)  "<BaseThrust>"
  FlightCommandFields/1 -> ControlDiagnosticPack/1(alt)  "<HeightReference>"
  ControlReferences/1 -> ControlReferencesFields/1
  FlightCommand/1 -> FlightCommandFields/1
  MotorDiagnostics/1 -> MotorDiagnosticsFields/1

== system HorizontalClosedLoop/FlightControl/TakeoffHoverControl/JapaneseExplanation ==

== system HorizontalClosedLoop/FlightControl/TakeoffHoverControl/MotorAllocation ==
  MotorEffort : Inport
  MotorContext : Inport  Port=2
  MotorCommandBus : BusCreator  Description=MotorCommandBus：異なる単位・型を持つ関連信号を名前付きバスにまとめます。入力線の信号名が項目名です。  Inputs=2
  MotorContextFields : BusSelector  Description=MotorContextFields：バスから ControlContext.Run,ControlContext.Reset,PilotInput.OverG,FlightContext.Branch,Dt を選びます。元のベクトルの成分順序は変更しません。  OutputSignals=ControlContext.Run,ControlContext.Reset,PilotInput.OverG,FlightContext.Branch,Dt
  MotorEffortFields : BusSelector  Description=MotorEffortFields：バスから Thrust,RollTorque,PitchTorque,YawTorque を選びます。元のベクトルの成分順序は変更しません。  OutputSignals=Thrust,RollTorque,PitchTorque,YawTorque
  MotorMixerFilter8bit : Subsystem  Description=4 モーターの符号付き配分、平滑化、飽和、8 bit 変換を一連の処理として示します。モーター順 [FR, FL, RR, RL] は出力・ログでも同じです。
      mask help: 4 モーターの符号付き配分、平滑化、飽和、8 bit 変換を一連の処理として示します。モーター順 [FR, FL, RR, RL] は出力・ログでも同じです。
      mask Display: disp('MotorMixerFilter8bit');port_label('input',1,'Thrust');port_label('input',2,'RollTorque');port_label('input',3,'PitchTorque');port_label('input',4,'YawTorque');port_label('input',5,'Run');port_label('input',6,'Reset');port_label('input',7,'OverG');port_label('input',8,'Mode');port_label('input',9,'Dt');port_label('output',1,'Duty4');port_label('output',2,'Counts4');port_label('output',3,'BeforeLimit4');
  MotorCommand : Outport
  BeforeLimit : Outport  Port=2
  wires:
  MotorCommandBus/1 -> MotorCommand/1  "MotorCommand"
  MotorMixerFilter8bit/2(Counts4) -> MotorCommandBus/2  "Counts"
  MotorMixerFilter8bit/1(Duty4) -> MotorCommandBus/1  "Duty"
  MotorContextFields/5 -> MotorMixerFilter8bit/9(Dt)  "<Dt>"
  MotorContextFields/4 -> MotorMixerFilter8bit/8(Mode)  "<Branch>"
  MotorContextFields/3 -> MotorMixerFilter8bit/7(OverG)  "<OverG>"
  MotorEffortFields/4 -> MotorMixerFilter8bit/4(YawTorque)  "<YawTorque>"
  MotorEffortFields/2 -> MotorMixerFilter8bit/2(RollTorque)  "<RollTorque>"
  MotorContextFields/1 -> MotorMixerFilter8bit/5(Run)  "<Run>"
  MotorContext/1 -> MotorContextFields/1
  MotorEffortFields/3 -> MotorMixerFilter8bit/3(PitchTorque)  "<PitchTorque>"
  MotorContextFields/2 -> MotorMixerFilter8bit/6(Reset)  "<Reset>"
  MotorEffort/1 -> MotorEffortFields/1
  MotorMixerFilter8bit/3(BeforeLimit4) -> BeforeLimit/1  "BeforeLimit"
  MotorEffortFields/1 -> MotorMixerFilter8bit/1(Thrust)  "<Thrust>"
